simulink model "TractorEnergyComputation"  (R2025a)
settings: Solver=ode23t  StartTime=0.0  StopTime=2200  RelTol=1e-3  AbsTol=1e-3
InitFcn:
  | TractorEnergyComputationInput
undefined symbols (not defined in the file): engine, implement, pump, tc, tire, tk, tphi, tykc, tykphi, tyn
libraries: nesl_utility x32, fl_lib x18, sdl_lib x6, simulink x5
(part 2 of 2)

== system TractorEnergyComputation/Tractor/Tire RL ==
  S : Inport
  Bus Selector : BusSelector  OutputSignals=Rear Right Tire.tykc,Rear Right Tire.tykphi,Rear Right Tire.tyn,Rear Right Tire.tk,Rear Right Tire.tphi,Rear Right Tire.tc
  PS Add : fl_lib/Physical Signals/Functions/PS Add
  PS Gain : fl_lib/Physical Signals/Functions/PS Gain  gain=0.5
  Simulink-PS Converter : nesl_utility/Simulink-PS Converter  PhysicalDomain=network_engine_domain  SubClassName=ps_input  LeftPortType=input  RightPortType=output  PseudoPeriodic=off  Frequencies=[]  NoiseDistribution=none  NoiseParameters=[]  Unit=kN/m^2  AffineConversion=off  FilteringAndDerivatives=provide  SimscapeFilterOrder=1  InputFilterTimeConstant=0.001  UdotUserProvided=0
  Simulink-PS Converter1 : nesl_utility/Simulink-PS Converter  PhysicalDomain=network_engine_domain  SubClassName=ps_input  LeftPortType=input  RightPortType=output  PseudoPeriodic=off  Frequencies=[]  NoiseDistribution=none  NoiseParameters=[]  Unit=deg  AffineConversion=off  FilteringAndDerivatives=provide  SimscapeFilterOrder=1  InputFilterTimeConstant=0.001  UdotUserProvided=0
  Simulink-PS Converter2 : nesl_utility/Simulink-PS Converter  PhysicalDomain=network_engine_domain  SubClassName=ps_input  LeftPortType=input  RightPortType=output  PseudoPeriodic=off  Frequencies=[]  NoiseDistribution=none  NoiseParameters=[]  Unit=cm  AffineConversion=off  FilteringAndDerivatives=provide  SimscapeFilterOrder=1  InputFilterTimeConstant=0.001  UdotUserProvided=0
  Simulink-PS Converter3 : nesl_utility/Simulink-PS Converter  PhysicalDomain=network_engine_domain  SubClassName=ps_input  LeftPortType=input  RightPortType=output  PseudoPeriodic=off  Frequencies=[]  NoiseDistribution=none  NoiseParameters=[]  Unit=1  AffineConversion=off  FilteringAndDerivatives=provide  SimscapeFilterOrder=1  InputFilterTimeConstant=0.001  UdotUserProvided=0
  Simulink-PS Converter4 : nesl_utility/Simulink-PS Converter  PhysicalDomain=network_engine_domain  SubClassName=ps_input  LeftPortType=input  RightPortType=output  PseudoPeriodic=off  Frequencies=[]  NoiseDistribution=none  NoiseParameters=[]  Unit=1  AffineConversion=off  FilteringAndDerivatives=provide  SimscapeFilterOrder=1  InputFilterTimeConstant=0.001  UdotUserProvided=0
  Simulink-PS Converter5 : nesl_utility/Simulink-PS Converter  PhysicalDomain=network_engine_domain  SubClassName=ps_input  LeftPortType=input  RightPortType=output  PseudoPeriodic=off  Frequencies=[]  NoiseDistribution=none  NoiseParameters=[]  Unit=1  AffineConversion=off  FilteringAndDerivatives=provide  SimscapeFilterOrder=1  InputFilterTimeConstant=0.001  UdotUserProvided=0
  Tire RL : SimscapeComponentBlock  SourceFile=tire_soil  ComponentPath=tire_soil  ComponentVariants="[\"tire_soil\"]"  ComponentVariantNames="[\"tire_soil\"]"  ClassName=tire_soil  SchemaVersion=1  load_TLU=tire.loadVector kN  p_inflation_TLU=tire.inflationPressureVector kPa  deflection_TLU="tire.deflectionTable  cm"  area_TLU=tire.contactPatchArea cm^2  inflation_pressure=tire.inflationPressure kPa  k_e=tire.constructionCoefficient  r_e=tire.rollingRadiusRear m  bti=tire.sectionWidth m  hti=tire.sectionHeight m  model_compliance=sdl.enum.compliance.off  stiffness=1e6 N/m  damping=1000 N*s/m  model_inertia=sdl.enum.model_inertia.off  inertia=2 kg*m^2  initial_velocity=0 rad/s  vxlow=1 m/s  v_tr_thr=0.001 m/s  kpumin=-1.5  kpumax=1.5  p_thr=0.01 bar  b_thr=1 mm  r_e_t=0.5 m  rolling_radius_model=sdl.enum.RollingRadiusParameterization.Constant  fz0=4000 N  r_0=0.5 m  breff=8.39  dreff=0.26  freff=0.074  q_re0=0.99  q_v1=0.008  longvl=17 m/s  cz=5e5 N/m
      settings: CopyFcn=simscape.sscblock.internal.componentBlockCallback(gcbh,'COPY')  PreCopyFcn=simscape.sscblock.internal.componentBlockCallback(gcbh,'PRECOPY')  PreDeleteFcn=simscape.sscblock.internal.componentBlockCallback(gcbh,'PREDELETE')  InternalSimscapePortConfiguration="{\"Bottom\":[{\"id\":\"tykc\",\"label\":\"tykc\",\"type\":\"input\"},{\"id\":\"tykphi\",\"label\":\"tykphi\",\"type\":\"input\"},{\"id\":\"tyn\",\"label\":\"tyn\",\"type\":\"input\"}],\"Left\":[{\"id\":\"A\",\"label\":\"A\",\"type\":\"foundation.mechanical.rotational.rotational\"},{\"id\":\"H\",\"label\":\"H\",\"type\":\"foundation.mechanical.translational.translational\"}],\"Right\":[{\"id\":\"S\",\"label\":\"S\",\"type\":\"output\"}],\"Top\":[{\"id\":\"N\",\"label\":\"N\",\"type\":\"input\"},{\"id\":\"tc\",\"label\":\"tc\",\"type\":\"input\"},{\"id\":\"tphi\",\"label\":\"tphi\",\"type\":\"input\"},{\"id\":\"tk\",\"label\":\"tk\",\"type\":\"input\"}]}"
      mask Type: Tire (Tire-Soil)
  H : PMIOPort  Side=Left
  N : PMIOPort  Port=2  Side=Left
  VF : PMIOPort  Port=3  Side=Right
  RLT : PMIOPort  Port=4  Side=Right
  wires:
  S/1 -> Bus Selector/1
  Bus Selector/3 -> Simulink-PS Converter3/1  "<tyn>"
  Bus Selector/2 -> Simulink-PS Converter4/1  "<tykphi>"
  Bus Selector/4 -> Simulink-PS Converter2/1  "<tk>"
  Bus Selector/5 -> Simulink-PS Converter1/1  "<tphi>"
  Bus Selector/1 -> Simulink-PS Converter5/1  "<tykc>"
  Bus Selector/6 -> Simulink-PS Converter/1  "<tc>"
  connections:
  Simulink-PS Converter/RConn1 -- Tire RL/LConn4
  Simulink-PS Converter2/RConn1 -- Tire RL/LConn6
  Simulink-PS Converter1/RConn1 -- Tire RL/LConn5
  Simulink-PS Converter3/RConn1 -- Tire RL/RConn4
  Simulink-PS Converter5/RConn1 -- Tire RL/RConn2
  Simulink-PS Converter4/RConn1 -- Tire RL/RConn3
  PS Add/LConn1 -- N/RConn1
  VF/RConn1 -- PS Gain/LConn1
  PS Gain/RConn1 -- PS Add/LConn2
  PS Add/RConn1 -- Tire RL/LConn3
  RLT/RConn1 -- Tire RL/LConn1
  H/RConn1 -- Tire RL/LConn2

== system TractorEnergyComputation/Tractor/Tire RR ==
  S : Inport
  Bus Selector : BusSelector  OutputSignals=Rear Left Tire.tykc,Rear Left Tire.tykphi,Rear Left Tire.tyn,Rear Left Tire.tk,Rear Left Tire.tphi,Rear Left Tire.tc
  PS Add : fl_lib/Physical Signals/Functions/PS Add
  PS Gain : fl_lib/Physical Signals/Functions/PS Gain  gain=0.5
  Simulink-PS Converter : nesl_utility/Simulink-PS Converter  PhysicalDomain=network_engine_domain  SubClassName=ps_input  LeftPortType=input  RightPortType=output  PseudoPeriodic=off  Frequencies=[]  NoiseDistribution=none  NoiseParameters=[]  Unit=kN/m^2  AffineConversion=off  FilteringAndDerivatives=provide  SimscapeFilterOrder=1  InputFilterTimeConstant=0.001  UdotUserProvided=0
  Simulink-PS Converter1 : nesl_utility/Simulink-PS Converter  PhysicalDomain=network_engine_domain  SubClassName=ps_input  LeftPortType=input  RightPortType=output  PseudoPeriodic=off  Frequencies=[]  NoiseDistribution=none  NoiseParameters=[]  Unit=deg  AffineConversion=off  FilteringAndDerivatives=provide  SimscapeFilterOrder=1  InputFilterTimeConstant=0.001  UdotUserProvided=0
  Simulink-PS Converter2 : nesl_utility/Simulink-PS Converter  PhysicalDomain=network_engine_domain  SubClassName=ps_input  LeftPortType=input  RightPortType=output  PseudoPeriodic=off  Frequencies=[]  NoiseDistribution=none  NoiseParameters=[]  Unit=cm  AffineConversion=off  FilteringAndDerivatives=provide  SimscapeFilterOrder=1  InputFilterTimeConstant=0.001  UdotUserProvided=0
  Simulink-PS Converter3 : nesl_utility/Simulink-PS Converter  PhysicalDomain=network_engine_domain  SubClassName=ps_input  LeftPortType=input  RightPortType=output  PseudoPeriodic=off  Frequencies=[]  NoiseDistribution=none  NoiseParameters=[]  Unit=1  AffineConversion=off  FilteringAndDerivatives=provide  SimscapeFilterOrder=1  InputFilterTimeConstant=0.001  UdotUserProvided=0
  Simulink-PS Converter4 : nesl_utility/Simulink-PS Converter  PhysicalDomain=network_engine_domain  SubClassName=ps_input  LeftPortType=input  RightPortType=output  PseudoPeriodic=off  Frequencies=[]  NoiseDistribution=none  NoiseParameters=[]  Unit=1  AffineConversion=off  FilteringAndDerivatives=provide  SimscapeFilterOrder=1  InputFilterTimeConstant=0.001  UdotUserProvided=0
  Simulink-PS Converter5 : nesl_utility/Simulink-PS Converter  PhysicalDomain=network_engine_domain  SubClassName=ps_input  LeftPortType=input  RightPortType=output  PseudoPeriodic=off  Frequencies=[]  NoiseDistribution=none  NoiseParameters=[]  Unit=1  AffineConversion=off  FilteringAndDerivatives=provide  SimscapeFilterOrder=1  InputFilterTimeConstant=0.001  UdotUserProvided=0
  Tire RR : SimscapeComponentBlock  SourceFile=tire_soil  ComponentPath=tire_soil  ComponentVariants="[\"tire_soil\"]"  ComponentVariantNames="[\"tire_soil\"]"  ClassName=tire_soil  SchemaVersion=1  load_TLU=tire.loadVector kN  p_inflation_TLU=tire.inflationPressureVector kPa  deflection_TLU=tire.deflectionTable cm  area_TLU=tire.contactPatchArea cm^2  inflation_pressure=tire.inflationPressure kPa  k_e=tire.constructionCoefficient  r_e=tire.rollingRadiusRear m  bti=tire.sectionWidth m  hti=tire.sectionHeight m  model_compliance=sdl.enum.compliance.off  stiffness=1e6 N/m  damping=1000 N*s/m  model_inertia=sdl.enum.model_inertia.off  inertia=2 kg*m^2  initial_velocity=0 rad/s  vxlow=1 m/s  v_tr_thr=0.001 m/s  kpumin=-1.5  kpumax=1.5  p_thr=0.01 bar  b_thr=1 mm  r_e_t=0.5 m  rolling_radius_model=sdl.enum.RollingRadiusParameterization.Constant  fz0=4000 N  r_0=0.5 m  breff=8.39  dreff=0.26  freff=0.074  q_re0=0.99  q_v1=0.008  longvl=17 m/s  cz=5e5 N/m
      settings: CopyFcn=simscape.sscblock.internal.componentBlockCallback(gcbh,'COPY')  PreCopyFcn=simscape.sscblock.internal.componentBlockCallback(gcbh,'PRECOPY')  PreDeleteFcn=simscape.sscblock.internal.componentBlockCallback(gcbh,'PREDELETE')  InternalSimscapePortConfiguration="{\"Bottom\":[{\"id\":\"tykc\",\"label\":\"tykc\",\"type\":\"input\"},{\"id\":\"tykphi\",\"label\":\"tykphi\",\"type\":\"input\"},{\"id\":\"tyn\",\"label\":\"tyn\",\"type\":\"input\"}],\"Left\":[{\"id\":\"A\",\"label\":\"A\",\"type\":\"foundation.mechanical.rotational.rotational\"},{\"id\":\"H\",\"label\":\"H\",\"type\":\"foundation.mechanical.translational.translational\"}],\"Right\":[{\"id\":\"S\",\"label\":\"S\",\"type\":\"output\"}],\"Top\":[{\"id\":\"N\",\"label\":\"N\",\"type\":\"input\"},{\"id\":\"tc\",\"label\":\"tc\",\"type\":\"input\"},{\"id\":\"tphi\",\"label\":\"tphi\",\"type\":\"input\"},{\"id\":\"tk\",\"label\":\"tk\",\"type\":\"input\"}]}"
      mask Type: Tire (Tire-Soil)
  N : PMIOPort  Side=Left
  H : PMIOPort  Port=2  Side=Left
  RRT : PMIOPort  Port=3  Side=Left
  VF : PMIOPort  Port=4  Side=Right
  wires:
  S/1 -> Bus Selector/1
  Bus Selector/6 -> Simulink-PS Converter/1  "<tc>"
  Bus Selector/1 -> Simulink-PS Converter5/1  "<tykc>"
  Bus Selector/2 -> Simulink-PS Converter4/1  "<tykphi>"
  Bus Selector/3 -> Simulink-PS Converter3/1  "<tyn>"
  Bus Selector/4 -> Simulink-PS Converter2/1  "<tk>"
  Bus Selector/5 -> Simulink-PS Converter1/1  "<tphi>"
  connections:
  Simulink-PS Converter/RConn1 -- Tire RR/LConn4
  Simulink-PS Converter1/RConn1 -- Tire RR/LConn5
  Simulink-PS Converter2/RConn1 -- Tire RR/LConn6
  Simulink-PS Converter3/RConn1 -- Tire RR/RConn4
  Simulink-PS Converter4/RConn1 -- Tire RR/RConn3
  Simulink-PS Converter5/RConn1 -- Tire RR/RConn2
  PS Gain/RConn1 -- PS Add/LConn2
  N/RConn1 -- PS Add/LConn1
  VF/RConn1 -- PS Gain/LConn1
  PS Add/RConn1 -- Tire RR/LConn3
  RRT/RConn1 -- Tire RR/LConn1
  H/RConn1 -- Tire RR/LConn2

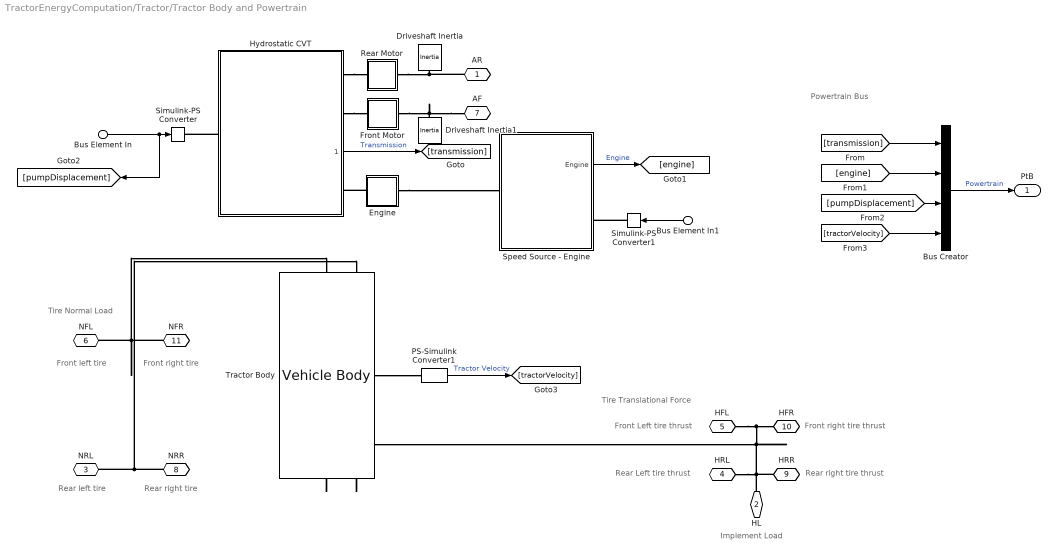
== system TractorEnergyComputation/Tractor/Tractor Body and Powertrain ==
  note: Powertrain Bus
  note: Tire Normal Load
  note: Tire Translational Force
  note: Front right tire thrust
  note: Rear right tire thrust
  note: Front Left tire thrust
  note: Rear Left tire thrust
  note: Front right tire
  note: Rear left tire
  note: Front left tire
  note: Rear right tire
  note: Implement Load
  Bus Element In : Inport  PortName=C  Element=Pump Displacement
  Bus Element In1 : Inport  PortName=C  Element=Speed Command
  Bus Creator : BusCreator  Inputs=4
  Driveshaft Inertia : fl_lib/Mechanical/Rotational Elements/Inertia  inertia=finalDrive.inertiaDriveshaft kg*m^2  num_ports=foundation.enum.numPorts2.one  w_specify=on  w_priority=None  w=0 rpm  w_nominal_specify=off  w_nominal_value=1  w_nominal_unit=rad/s  t_specify=off  t_priority=High  t=0 N*m  t_nominal_specify=off  t_nominal_value=1  t_nominal_unit=N*m
  Driveshaft Inertia1 : fl_lib/Mechanical/Rotational Elements/Inertia  inertia=finalDrive.inertiaDriveshaft kg*m^2  num_ports=foundation.enum.numPorts2.one  w_specify=on  w_priority=None  w=0 rpm  w_nominal_specify=off  w_nominal_value=1  w_nominal_unit=rad/s  t_specify=off  t_priority=High  t=0 N*m  t_nominal_specify=off  t_nominal_value=1  t_nominal_unit=N*m
  Engine : Subsystem
      settings: PortSchema="{\"entries\":[{\"content\":{\"sides\":[{\"content\":{},\"type\":\"ConnectorPlacement.EquallySpacedRectSide\",\"uuid\":\"92eebf28-269a-4925-a955-a9d1c44b965b\"},{\"content\":{\"side\":\"RIGHT\"},\"type\":\"ConnectorPlacement.EquallySpacedRectSide\",\"uuid\":\"c7d6808e-0022-4ac6-baaf-1452e02bfec1\"},{\"content\":{\"connectorIds\":[\"LConn1\"],\"side\":\"TOP\"},\"type\":\"ConnectorPlacement.EquallySpacedRectSide\",\"uuid\":\"598768ff-2342-4a1c-9a1c-354d4df076d5\"},{\"content\":{\"connectorIds\":[\"RConn1\"],\"side\":\"BOTTOM\"},\"type\":\"ConnectorPlacement.EquallySpacedRectSide\",\"uuid\":\"a8e2d810-51b4-480a-8888-7fbba5dd7c90\"}]},\"type\":\"ConnectorPlacement.EquallySpacedConnector\",\"uuid\":\"c2f50c2b-379b-41d6-9ef6-b6270bc7ebba\"}],\"packageUris\":[\"http://schema.mathworks.com/mf0/Connector/R2020b\"],\"version\":\"1.0\"}"
  Front Motor : Subsystem
      settings: PortSchema="{\"entries\":[{\"content\":{\"sides\":[{\"content\":{},\"type\":\"ConnectorPlacement.EquallySpacedRectSide\",\"uuid\":\"92eebf28-269a-4925-a955-a9d1c44b965b\"},{\"content\":{\"side\":\"RIGHT\"},\"type\":\"ConnectorPlacement.EquallySpacedRectSide\",\"uuid\":\"c7d6808e-0022-4ac6-baaf-1452e02bfec1\"},{\"content\":{\"connectorIds\":[\"LConn1\"],\"side\":\"TOP\"},\"type\":\"ConnectorPlacement.EquallySpacedRectSide\",\"uuid\":\"598768ff-2342-4a1c-9a1c-354d4df076d5\"},{\"content\":{\"connectorIds\":[\"RConn1\"],\"side\":\"BOTTOM\"},\"type\":\"ConnectorPlacement.EquallySpacedRectSide\",\"uuid\":\"a8e2d810-51b4-480a-8888-7fbba5dd7c90\"}]},\"type\":\"ConnectorPlacement.EquallySpacedConnector\",\"uuid\":\"c2f50c2b-379b-41d6-9ef6-b6270bc7ebba\"}],\"packageUris\":[\"http://schema.mathworks.com/mf0/Connector/R2020b\"],\"version\":\"1.0\"}"
  Hydrostatic CVT : Subsystem  ReferencedSubsystem=HydrostaticCVT
      settings: PortSchema="{\"entries\":[{\"content\":{\"sides\":[{\"content\":{\"connectorIds\":[\"LConn2\"]},\"type\":\"ConnectorPlacement.EquallySpacedRectSide\",\"uuid\":\"e98c307e-384f-4f6d-84ec-b1e3747c2742\"},{\"content\":{\"connectorIds\":[\"RConn1\",\"RConn2\",\"Out1\",\"LConn1\"],\"side\":\"RIGHT\"},\"type\":\"ConnectorPlacement.EquallySpacedRectSide\",\"uuid\":\"8cf92fb4-b64d-4865-8313-0964738a3102\"},{\"content\":{\"side\":\"TOP\"},\"type\":\"ConnectorPlacement.EquallySpacedRectSide\",\"uuid\":\"5529046d-fa81-4c87-9e58-4bcc6f8343df\"},{\"content\":{\"side\":\"BOTTOM\"},\"type\":\"ConnectorPlacement.EquallySpacedRectSide\",\"uuid\":\"0f2d78cd-5597-48dc-a814-c7cd3f15dde1\"}]},\"type\":\"ConnectorPlacement.EquallySpacedConnector\",\"uuid\":\"d1cf8514-964a-4874-a812-4541b3ddd120\"}],\"packageUris\":[\"http://schema.mathworks.com/mf0/Connector/R2020b\"],\"version\":\"1.0\"}"
  PS-Simulink Converter1 : nesl_utility/PS-Simulink Converter  PhysicalDomain=network_engine_domain  SubClassName=ps_output  LeftPortType=input  RightPortType=output  PseudoPeriodic=off  Frequencies=[]  VectorFormat=1-D array  Unit=km/hr  AffineConversion=off
  Rear Motor : Subsystem
      settings: PortSchema="{\"entries\":[{\"content\":{\"sides\":[{\"content\":{},\"type\":\"ConnectorPlacement.EquallySpacedRectSide\",\"uuid\":\"92eebf28-269a-4925-a955-a9d1c44b965b\"},{\"content\":{\"side\":\"RIGHT\"},\"type\":\"ConnectorPlacement.EquallySpacedRectSide\",\"uuid\":\"c7d6808e-0022-4ac6-baaf-1452e02bfec1\"},{\"content\":{\"connectorIds\":[\"LConn1\"],\"side\":\"TOP\"},\"type\":\"ConnectorPlacement.EquallySpacedRectSide\",\"uuid\":\"598768ff-2342-4a1c-9a1c-354d4df076d5\"},{\"content\":{\"connectorIds\":[\"RConn1\"],\"side\":\"BOTTOM\"},\"type\":\"ConnectorPlacement.EquallySpacedRectSide\",\"uuid\":\"a8e2d810-51b4-480a-8888-7fbba5dd7c90\"}]},\"type\":\"ConnectorPlacement.EquallySpacedConnector\",\"uuid\":\"c2f50c2b-379b-41d6-9ef6-b6270bc7ebba\"}],\"packageUris\":[\"http://schema.mathworks.com/mf0/Connector/R2020b\"],\"version\":\"1.0\"}"
  Simulink-PS Converter : nesl_utility/Simulink-PS Converter  PhysicalDomain=network_engine_domain  SubClassName=ps_input  LeftPortType=input  RightPortType=output  PseudoPeriodic=off  Frequencies=[]  NoiseDistribution=none  NoiseParameters=[]  Unit=cm^3/rev  AffineConversion=off  FilteringAndDerivatives=provide  SimscapeFilterOrder=1  InputFilterTimeConstant=0.001  UdotUserProvided=0
  Simulink-PS Converter1 : nesl_utility/Simulink-PS Converter  PhysicalDomain=network_engine_domain  SubClassName=ps_input  LeftPortType=input  RightPortType=output  PseudoPeriodic=off  Frequencies=[]  NoiseDistribution=none  NoiseParameters=[]  Unit=rpm  AffineConversion=off  FilteringAndDerivatives=provide  SimscapeFilterOrder=1  InputFilterTimeConstant=0.001  UdotUserProvided=0
  Speed Source - Engine : Subsystem
      settings: PortSchema="{\"entries\":[{\"content\":{\"sides\":[{\"content\":{\"connectorIds\":[\"Out1\",\"LConn1\"]},\"type\":\"ConnectorPlacement.EquallySpacedRectSide\",\"uuid\":\"893d34ea-3b68-4e33-a67a-452726c44412\"},{\"content\":{\"connectorIds\":[\"RConn1\"],\"side\":\"RIGHT\"},\"type\":\"ConnectorPlacement.EquallySpacedRectSide\",\"uuid\":\"36b2695b-8811-427c-b3d4-10ce1d3bb3e5\"},{\"content\":{\"side\":\"TOP\"},\"type\":\"ConnectorPlacement.EquallySpacedRectSide\",\"uuid\":\"39e3a5de-3435-43d6-80cb-ad06275add25\"}]},\"type\":\"ConnectorPlacement.EquallySpacedConnector\",\"uuid\":\"b2b9cbdb-1a63-4aca-a9b5-b09fdbada543\"}],\"packageUris\":[\"http://schema.mathworks.com/mf0/Connector/R2020b\"],\"version\":\"1.0\"}"
  Tractor Body : sdl_lib/Tires & Vehicles/Vehicle Body  mass=driveline.massTractor kg  n_w=driveline.nWheelsPerAxle  x_f=driveline.distanceFrontAxleCG m  x_r=driveline.distanceRearAxleCG m  y_c=driveline.heightCG m  mass_var=simscape.enum.onoff.off  g=9.81 m/s^2  liftoff_warning=simscape.enum.onoff.off  area=driveline.areaFrontal m^2  Cd_var=false  Cd=driveline.coefficientDrag  rho=driveline.densityAir kg/m^3  model_pitch=simscape.enum.onoff.off  inertia=4000 kg*m^2  suspension_model=sdl.enum.linearTLU.linear  k_f=1e4 N/m  b_f=1e4 N/(m/s)  k_r=1e4 N/m  b_r=1e4 N/(m/s)  k_f_TLU=[-2000, -1000, 0, 1000, 2000] N  x_f_TLU=[-.4, -.2, 0, .2, .4] m  b_f_TLU=[-200, -100, 0, 100, 200] N  v_f_TLU=[-4, -2, 0, 2, 4] m/s  k_r_TLU=[-2000, -1000, 0, 1000, 2000] N  x_r_TLU=[-.4, -.2, 0, .2, .4] m  b_r_TLU=[-200, -100, 0, 100, 200] N  v_r_TLU=[-4, -2, 0, 2, 4] m/s  interp_method=simscape.enum.interpolation.linear  extrap_method=simscape.enum.extrapolation.linear  model_hardstop=simscape.enum.onoff.off  upper_bound_f=.25 m  lower_bound_f=-.25 m  stop_k_f=1e6 N/m  stop_b_f=150 N/(m/s)  upper_bound_r=.25 m  lower_bound_r=-.25 m  stop_k_r=1e6 N/m  stop_b_r=150 N/(m/s)  initial_pitch=0 rad  initial_pitch_rate=0 rad/s  v_specify=off  v_priority=High  v=0 m/s  v_nominal_specify=off  v_nominal_value=1  v_nominal_unit=m/s
      settings: InternalSimscapePortConfiguration="{\"Bottom\":[{\"id\":\"NR\",\"label\":\"NR\",\"type\":\"output\"},{\"id\":\"NF\",\"label\":\"NF\",\"type\":\"output\"},{\"id\":\"beta\",\"label\":\"beta\",\"type\":\"input\"}],\"Left\":[{\"id\":\"H\",\"label\":\"H\",\"type\":\"foundation.mechanical.translational.translational\"}],\"Right\":[],\"Top\":[{\"id\":\"V\",\"label\":\"V\",\"type\":\"output\"},{\"id\":\"wind\",\"label\":\"W\",\"type\":\"input\"}]}"
  AR : PMIOPort  Side=Left
  HL : PMIOPort  Port=2  Side=Left
  NRL : PMIOPort  Port=3  Side=Left
  HRL : PMIOPort  Port=4  Side=Left
  HFL : PMIOPort  Port=5  Side=Left
  NFL : PMIOPort  Port=6  Side=Left
  "AF " : PMIOPort  Port=7  Side=Right
  NRR : PMIOPort  Port=8  Side=Right
  HRR : PMIOPort  Port=9  Side=Right
  HFR : PMIOPort  Port=10  Side=Right
  NFR : PMIOPort  Port=11  Side=Right
  PtB : Outport
  wires:
  PS-Simulink Converter1/1 -> [tractorVelocity]  "Tractor Velocity"
  Hydrostatic CVT/1 -> [transmission]  "Transmission"
  Speed Source - Engine/1(Engine) -> [engine]  "Engine"
  Bus Creator/1 -> PtB/1  "Powertrain"
  [transmission] -> Bus Creator/1
  [engine] -> Bus Creator/2
  [pumpDisplacement] -> Bus Creator/3
  [tractorVelocity] -> Bus Creator/4
  Bus Element In/1 -> [pumpDisplacement], Simulink-PS Converter/1
  Bus Element In1/1 -> Simulink-PS Converter1/1
  connections:
  HRL/RConn1 -- HL/RConn1 -- HRR/RConn1 -- HFL/RConn1 -- HFR/RConn1 -- Tractor Body/LConn1
  AR/RConn1 -- Rear Motor/RConn1 -- Driveshaft Inertia/LConn1
  Engine/LConn1 -- Speed Source - Engine/RConn1
  NRR/RConn1 -- Tractor Body/RConn1 -- NRL/RConn1
  NFR/RConn1 -- Tractor Body/RConn2 -- NFL/RConn1
  Tractor Body/LConn2 -- PS-Simulink Converter1/LConn1
  Hydrostatic CVT/LConn2 -- Simulink-PS Converter/RConn1
  "AF "/RConn1 -- Front Motor/RConn1 -- Driveshaft Inertia1/LConn1
  Simulink-PS Converter1/RConn1 -- Speed Source - Engine/LConn1
  Hydrostatic CVT/RConn1 -- Rear Motor/LConn1
  Hydrostatic CVT/RConn2 -- Front Motor/LConn1
  Engine/RConn1 -- Hydrostatic CVT/LConn1

== system TractorEnergyComputation/System Signals and Information/Power and Energy Calculations/Charge Pump Computation ==
  System Bus : Inport
  Bus Selector : BusSelector  OutputSignals=Engine.engineSpeed,Transmission.Charge Pump.trq (N*m),Pump Displacement
  Bus Selector1 : BusSelector  OutputSignals=Pump Displacement,Transmission.Charge Pump.q (m^3/s),Transmission.Charge Pump.P (bar)
  Charge Pump Input Energy Computation : Subsystem
  Charge Pump Output Energy Computation : Subsystem
  Sump open pressure : Constant  Value=1.01325
  Input Energy : Outport
  "Output Energy " : Outport  Port=2
  Input Power : Outport  Port=3
  Output Power : Outport  Port=4
  wires:
  Charge Pump Output Energy Computation/1(Output Energy) -> "Output Energy "/1
  Charge Pump Input Energy Computation/1(Input Energy) -> Input Energy/1
  Bus Selector1/3 -> Charge Pump Output Energy Computation/3(pressureB (bar))  "<P (bar)>"
  Bus Selector1/2 -> Charge Pump Output Energy Computation/2(pumpFlow (m^3/s))  "<q (m^3/s)>"
  Bus Selector1/1 -> Charge Pump Output Energy Computation/1(dispPump (cm^3/rev))  "<Pump Displacement>"
  Bus Selector/3 -> Charge Pump Input Energy Computation/3(dispPump (cm^3/rev))  "<Pump Displacement>"
  Bus Selector/2 -> Charge Pump Input Energy Computation/2(tPump (N*m))  "<trq (N*m)>"
  Bus Selector/1 -> Charge Pump Input Energy Computation/1(wEngine (rpm))  "<engineSpeed>"
  System Bus/1 -> Bus Selector/1, Bus Selector1/1
  Sump open pressure/1 -> Charge Pump Output Energy Computation/4(pressureA (bar))
  Charge Pump Input Energy Computation/2(Input Power) -> Input Power/1
  Charge Pump Output Energy Computation/2(Output Power) -> Output Power/1

== system TractorEnergyComputation/System Signals and Information/Power and Energy Calculations/Front Motor Computation ==
  System Bus : Inport
  Bus Selector : BusSelector  OutputSignals=Transmission.Front Motor.w (rpm),Transmission.Front Motor.trq (N*m),Pump Displacement
  Bus Selector1 : BusSelector  OutputSignals=Pump Displacement,Transmission.Front Motor.q (m^3/s),Transmission.Pipe A.pB (bar),Transmission.Pipe B.pB (bar)
  Motor Input Energy Computation : Subsystem
  Motor Output Energy Computation : Subsystem
  Output Energy : Outport
  "Input Energy " : Outport  Port=2
  Output Power : Outport  Port=3
  Input Power : Outport  Port=4
  wires:
  Bus Selector1/4 -> Motor Input Energy Computation/4(pressureB (bar))  "<pB (bar)>"
  Bus Selector1/3 -> Motor Input Energy Computation/3(pressureA (bar))  "<pB (bar)>"
  Bus Selector1/2 -> Motor Input Energy Computation/2(motorFlow (m^3/s))  "<q (m^3/s)>"
  Bus Selector1/1 -> Motor Input Energy Computation/1(dispPump (cm^3/rev))  "<Pump Displacement>"
  Bus Selector/1 -> Motor Output Energy Computation/1(wTransmission (rpm))  "<w (rpm)>"
  Bus Selector/3 -> Motor Output Energy Computation/3(dispPump (cm^3/rev))  "<Pump Displacement>"
  Bus Selector/2 -> Motor Output Energy Computation/2(tTransmission (N*m))  "<trq (N*m)>"
  System Bus/1 -> Bus Selector/1, Bus Selector1/1
  Motor Input Energy Computation/1("Input Energy ") -> "Input Energy "/1
  Motor Output Energy Computation/1(Output Energy) -> Output Energy/1
  Motor Output Energy Computation/2(Output Power) -> Output Power/1
  Motor Input Energy Computation/2(Input Power) -> Input Power/1

== system TractorEnergyComputation/System Signals and Information/Power and Energy Calculations/Pump Computation ==
  System Bus : Inport
  Bus Selector : BusSelector  OutputSignals=Engine.engineSpeed,Transmission.Main Pump.trq (N*m),Pump Displacement
  Bus Selector1 : BusSelector  OutputSignals=Pump Displacement,Transmission.Main Pump.q (m^3/s),Transmission.Pipe B.pA (bar),Transmission.Pipe A.pA (bar)
  Pump Input Energy Computation : Subsystem
  Pump Output Energy Computation : Subsystem
  Input Energy : Outport
  "Output Energy " : Outport  Port=2
  Input Power : Outport  Port=3
  Output Power : Outport  Port=4
  wires:
  System Bus/1 -> Bus Selector1/1, Bus Selector/1
  Bus Selector/1 -> Pump Input Energy Computation/1(wEngine (rpm))  "<engineSpeed>"
  Bus Selector/2 -> Pump Input Energy Computation/2(tPump (N*m))  "<trq (N*m)>"
  Bus Selector/3 -> Pump Input Energy Computation/3(dispPump (cm^3/rev))  "<Pump Displacement>"
  Bus Selector1/1 -> Pump Output Energy Computation/1(dispPump (cm^3/rev))  "<Pump Displacement>"
  Bus Selector1/2 -> Pump Output Energy Computation/2(pumpFlow (m^3/s))  "<q (m^3/s)>"
  Bus Selector1/3 -> Pump Output Energy Computation/3(pressureA (bar))  "<pA (bar)>"
  Bus Selector1/4 -> Pump Output Energy Computation/4(pressureB (bar))  "<pA (bar)>"
  Pump Input Energy Computation/1(Input Energy) -> Input Energy/1
  Pump Output Energy Computation/1(Output Energy) -> "Output Energy "/1
  Pump Input Energy Computation/2(Input Power) -> Input Power/1
  Pump Output Energy Computation/2(Output Power) -> Output Power/1

== system TractorEnergyComputation/System Signals and Information/Power and Energy Calculations/Rear Motor Computation ==
  System Bus : Inport
  Bus Selector : BusSelector  OutputSignals=Transmission.Rear Motor.w (rpm),Transmission.Rear Motor.trq (N*m),Pump Displacement
  Bus Selector1 : BusSelector  OutputSignals=Pump Displacement,Transmission.Rear Motor.q (m^3/s),Transmission.Pipe A.pB (bar),Transmission.Pipe B.pB (bar)
  Motor Input Energy Computation : Subsystem
  Motor Output Energy Computation : Subsystem
  Output Energy : Outport
  "Input Energy  " : Outport  Port=2
  Output Power : Outport  Port=3
  Input Power : Outport  Port=4
  wires:
  Motor Output Energy Computation/1(Output Energy) -> Output Energy/1
  Motor Input Energy Computation/1("Input Energy ") -> "Input Energy  "/1
  System Bus/1 -> Bus Selector1/1, Bus Selector/1
  Bus Selector/2 -> Motor Output Energy Computation/2(tTransmission (N*m))  "<trq (N*m)>"
  Bus Selector/3 -> Motor Output Energy Computation/3(dispPump (cm^3/rev))  "<Pump Displacement>"
  Bus Selector/1 -> Motor Output Energy Computation/1(wTransmission (rpm))  "<w (rpm)>"
  Bus Selector1/1 -> Motor Input Energy Computation/1(dispPump (cm^3/rev))  "<Pump Displacement>"
  Bus Selector1/2 -> Motor Input Energy Computation/2(motorFlow (m^3/s))  "<q (m^3/s)>"
  Bus Selector1/3 -> Motor Input Energy Computation/3(pressureA (bar))  "<pB (bar)>"
  Bus Selector1/4 -> Motor Input Energy Computation/4(pressureB (bar))  "<pB (bar)>"
  Motor Output Energy Computation/2(Output Power) -> Output Power/1
  Motor Input Energy Computation/2(Input Power) -> Input Power/1

== system TractorEnergyComputation/System Signals and Information/Power and Energy Calculations/Relief Valve A Computation ==
  System Bus : Inport
  Abs : Abs  ZeroCross=off  SaturateOnIntegerOverflow=off
  Abs1 : Abs  ZeroCross=off  SaturateOnIntegerOverflow=off
  Add1 : Sum  Inputs=+-
  Add2 : Sum  Inputs=+-
  Bus Selector : BusSelector  OutputSignals=Transmission.Pipe A.pB (bar),Transmission.Flow Relief A.q (m^3/s),Transmission.Pipe B.pB (bar)
  Gain1 : Gain  Gain=1e5
  Gain2 : Gain  Gain=1e5
  Integrator : Integrator
  Integrator1 : Integrator
  Product : Product
  Product1 : Product
  convert to kW : Gain  Gain=1e-3
  convert to kW1 : Gain  Gain=1e-3
  "Energy Loss " : Outport
  Power Loss : Outport  Port=2
  wires:
  Gain2/1 -> Abs/1
  Product/1 -> Gain2/1
  Product1/1 -> Gain1/1
  Gain1/1 -> Abs1/1
  Abs/1 -> convert to kW/1
  Abs1/1 -> convert to kW1/1
  Integrator/1 -> Add1/1  "Relief A Inlet Energy"
  Integrator1/1 -> Add1/2  "Relief A Outlet Energy"
  Add1/1 -> "Energy Loss "/1  "Energy Loss Relief Valve A"
  convert to kW/1 -> Add2/1, Integrator/1
  convert to kW1/1 -> Add2/2, Integrator1/1
  System Bus/1 -> Bus Selector/1
  Bus Selector/1 -> Product/1  "<pB (bar)>"
  Bus Selector/2 -> Product1/1, Product/2  "<q (m^3/s)>"
  Bus Selector/3 -> Product1/2  "<pB (bar)>"
  Add2/1 -> Power Loss/1  "Power Loss Relief Valve A"

== system TractorEnergyComputation/System Signals and Information/Power and Energy Calculations/Relief Valve B Computation ==
  System Bus : Inport
  Abs : Abs  ZeroCross=off  SaturateOnIntegerOverflow=off
  Abs1 : Abs  ZeroCross=off  SaturateOnIntegerOverflow=off
  Add1 : Sum  Inputs=-+
  Add2 : Sum  Inputs=-+
  Bus Selector : BusSelector  OutputSignals=Transmission.Pipe A.pB (bar),Transmission.Flow Relief B.q (m^3/s),Transmission.Pipe B.pB (bar)
  Gain1 : Gain  Gain=1e5
  Gain2 : Gain  Gain=1e5
  Integrator : Integrator
  Integrator1 : Integrator
  Product : Product
  Product1 : Product
  convert to kW : Gain  Gain=1e-3
  convert to kW1 : Gain  Gain=1e-3
  "Energy Loss " : Outport
  "Power Loss " : Outport  Port=2
  wires:
  Add1/1 -> "Energy Loss "/1  "Energy Loss Relief Valve B"
  Integrator1/1 -> Add1/2  "Relief B Inlet Energy"
  Integrator/1 -> Add1/1  "Relief B Outlet Energy"
  Abs1/1 -> convert to kW1/1
  Abs/1 -> convert to kW/1
  Gain1/1 -> Abs1/1
  Gain2/1 -> Abs/1
  convert to kW/1 -> Add2/1, Integrator/1
  System Bus/1 -> Bus Selector/1
  Bus Selector/1 -> Product/1  "<pB (bar)>"
  Bus Selector/3 -> Product1/2  "<pB (bar)>"
  Bus Selector/2 -> Product/2, Product1/1  "<q (m^3/s)>"
  Product/1 -> Gain2/1
  Product1/1 -> Gain1/1
  convert to kW1/1 -> Add2/2, Integrator1/1
  Add2/1 -> "Power Loss "/1  "Power Loss Relief Valve B"

== system TractorEnergyComputation/Tractor/Tractor Body and Powertrain/Engine ==
  Mechanical Rotational Reference : fl_lib/Mechanical/Rotational Elements/Mechanical Rotational Reference
  PS Terminator : fl_lib/Physical Signals/Sinks/PS Terminator
  Rotational Power Sensor : sdl_lib/Sensors/Rotational Power Sensor  measurement_type=sdl.enum.rotationalPowerSensorType.instantaneous  averaging_period=1 s  max_frequency=1000 Hz  max_speed=1000 rpm
      settings: InternalSimscapePortConfiguration="{\"Bottom\":[],\"Left\":[{\"id\":\"S\",\"label\":\"S\",\"type\":\"foundation.mechanical.rotational.rotational\"},{\"id\":\"R\",\"label\":\"R\",\"type\":\"foundation.mechanical.rotational.rotational\"},{\"id\":\"C\",\"label\":\"C\",\"type\":\"foundation.mechanical.rotational.rotational\"}],\"Right\":[{\"id\":\"P\",\"label\":\"P\",\"type\":\"output\"}],\"Top\":[]}"
  S : PMIOPort  Side=Left
  R : PMIOPort  Port=2  Side=Right
  connections:
  Rotational Power Sensor/RConn1 -- PS Terminator/LConn1
  Rotational Power Sensor/LConn3 -- Mechanical Rotational Reference/LConn1
  S/RConn1 -- Rotational Power Sensor/LConn1
  R/RConn1 -- Rotational Power Sensor/LConn2

== system TractorEnergyComputation/Tractor/Tractor Body and Powertrain/Front Motor ==
  Mechanical Rotational Reference : fl_lib/Mechanical/Rotational Elements/Mechanical Rotational Reference
  PS Terminator : fl_lib/Physical Signals/Sinks/PS Terminator
  Rotational Power Sensor : sdl_lib/Sensors/Rotational Power Sensor  measurement_type=sdl.enum.rotationalPowerSensorType.instantaneous  averaging_period=1 s  max_frequency=1000 Hz  max_speed=1000 rpm
      settings: InternalSimscapePortConfiguration="{\"Bottom\":[],\"Left\":[{\"id\":\"S\",\"label\":\"S\",\"type\":\"foundation.mechanical.rotational.rotational\"},{\"id\":\"R\",\"label\":\"R\",\"type\":\"foundation.mechanical.rotational.rotational\"},{\"id\":\"C\",\"label\":\"C\",\"type\":\"foundation.mechanical.rotational.rotational\"}],\"Right\":[{\"id\":\"P\",\"label\":\"P\",\"type\":\"output\"}],\"Top\":[]}"
  S : PMIOPort  Side=Left
  R : PMIOPort  Port=2  Side=Right
  connections:
  R/RConn1 -- Rotational Power Sensor/LConn2
  S/RConn1 -- Rotational Power Sensor/LConn1
  Rotational Power Sensor/LConn3 -- Mechanical Rotational Reference/LConn1
  Rotational Power Sensor/RConn1 -- PS Terminator/LConn1

== system TractorEnergyComputation/Tractor/Tractor Body and Powertrain/Rear Motor ==
  Mechanical Rotational Reference : fl_lib/Mechanical/Rotational Elements/Mechanical Rotational Reference
  PS Terminator : fl_lib/Physical Signals/Sinks/PS Terminator
  Rotational Power Sensor : sdl_lib/Sensors/Rotational Power Sensor  measurement_type=sdl.enum.rotationalPowerSensorType.instantaneous  averaging_period=1 s  max_frequency=1000 Hz  max_speed=1000 rpm
      settings: InternalSimscapePortConfiguration="{\"Bottom\":[],\"Left\":[{\"id\":\"S\",\"label\":\"S\",\"type\":\"foundation.mechanical.rotational.rotational\"},{\"id\":\"R\",\"label\":\"R\",\"type\":\"foundation.mechanical.rotational.rotational\"},{\"id\":\"C\",\"label\":\"C\",\"type\":\"foundation.mechanical.rotational.rotational\"}],\"Right\":[{\"id\":\"P\",\"label\":\"P\",\"type\":\"output\"}],\"Top\":[]}"
  S : PMIOPort  Side=Left
  R : PMIOPort  Port=2  Side=Right
  connections:
  Rotational Power Sensor/RConn1 -- PS Terminator/LConn1
  Rotational Power Sensor/LConn3 -- Mechanical Rotational Reference/LConn1
  S/RConn1 -- Rotational Power Sensor/LConn1
  R/RConn1 -- Rotational Power Sensor/LConn2

== system TractorEnergyComputation/Tractor/Tractor Body and Powertrain/Speed Source - Engine ==
  note: This tractor engine operates ar fixed speed through governor control for agriculture hydraulic equipment requirement.
      | The governor controls the fuel injection into the cylinders to maintain
      | speed constant to compensate for load.
  Ideal Angular Velocity Source : fl_lib/Mechanical/Mechanical Sources/Ideal Angular Velocity Source
  Mechanical Rotational Reference : fl_lib/Mechanical/Rotational Elements/Mechanical Rotational Reference
  Sensor Engine : Subsystem
      mask Display: disp('S')
  SC : PMIOPort  Side=Left
  Shaft : PMIOPort  Port=2  Side=Right
  Engine : Outport
  wires:
  Sensor Engine/1(engine) -> Engine/1
  connections:
  Mechanical Rotational Reference/LConn1 -- Ideal Angular Velocity Source/RConn2
  Ideal Angular Velocity Source/LConn1 -- Sensor Engine/LConn1
  Sensor Engine/RConn1 -- Shaft/RConn1
  Ideal Angular Velocity Source/RConn1 -- SC/RConn1

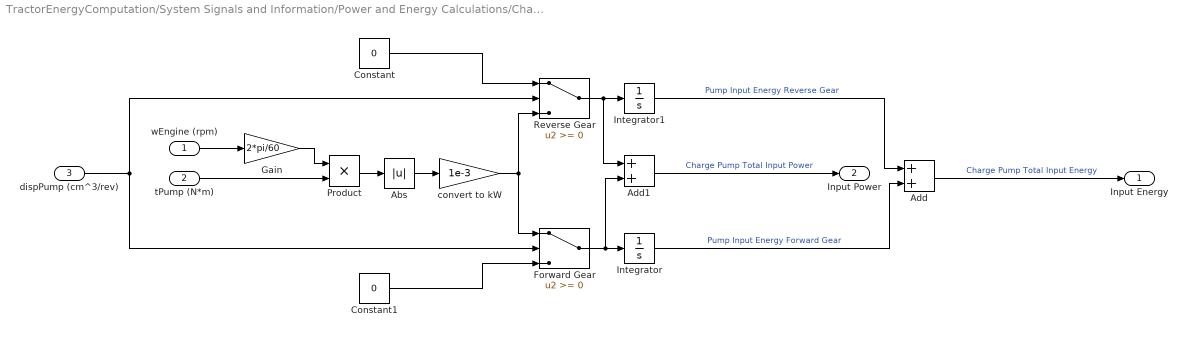
== system TractorEnergyComputation/System Signals and Information/Power and Energy Calculations/Charge Pump Computation/Charge Pump Input Energy Computation ==
  wEngine (rpm) : Inport
  tPump (N*m) : Inport  Port=2
  dispPump (cm^3/rev) : Inport  Port=3
  Abs : Abs  ZeroCross=off  SaturateOnIntegerOverflow=off
  Add : Sum
  Add1 : Sum
  Constant : Constant  Value=0
  Constant1 : Constant  Value=0
  Forward Gear : Switch  SaturateOnIntegerOverflow=off  InputSameDT=off
  Gain : Gain  Gain=2*pi/60
  Integrator : Integrator
  Integrator1 : Integrator
  Product : Product
  Reverse Gear : Switch  SaturateOnIntegerOverflow=off  InputSameDT=off
  convert to kW : Gain  Gain=1e-3
  Input Energy : Outport
  Input Power : Outport  Port=2
  wires:
  convert to kW/1 -> Reverse Gear/3, Forward Gear/1
  Abs/1 -> convert to kW/1
  Product/1 -> Abs/1
  Add/1 -> Input Energy/1  "Charge Pump Total Input Energy"
  Integrator/1 -> Add/2  "Pump Input Energy Forward Gear"
  Integrator1/1 -> Add/1  "Pump Input Energy Reverse Gear"
  Forward Gear/1 -> Add1/2, Integrator/1
  Reverse Gear/1 -> Add1/1, Integrator1/1
  Constant1/1 -> Forward Gear/3
  Constant/1 -> Reverse Gear/1
  dispPump (cm^3/rev)/1 -> Reverse Gear/2, Forward Gear/2
  wEngine (rpm)/1 -> Gain/1
  tPump (N*m)/1 -> Product/2
  Gain/1 -> Product/1
  Add1/1 -> Input Power/1  "Charge Pump Total Input Power"

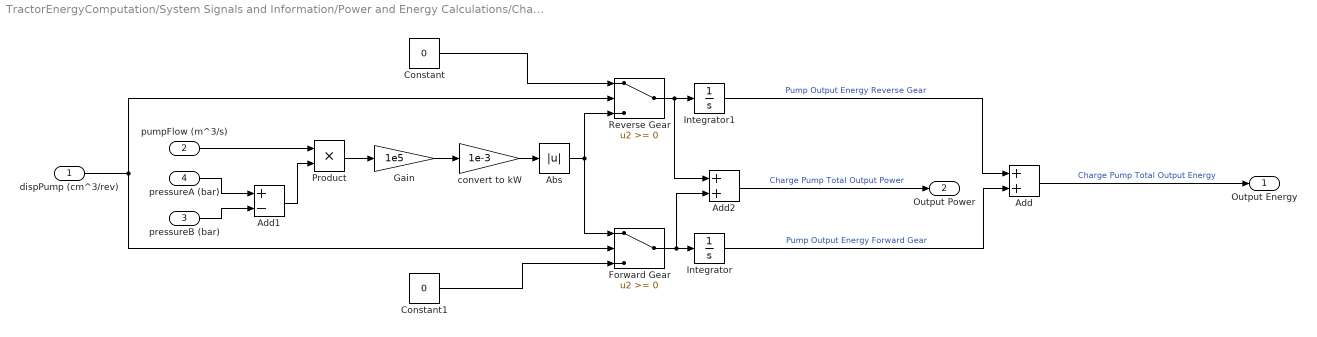
== system TractorEnergyComputation/System Signals and Information/Power and Energy Calculations/Charge Pump Computation/Charge Pump Output Energy Computation ==
  dispPump (cm^3/rev) : Inport
  pumpFlow (m^3/s) : Inport  Port=2
  pressureB (bar) : Inport  Port=3
  pressureA (bar) : Inport  Port=4
  Abs : Abs  ZeroCross=off  SaturateOnIntegerOverflow=off
  Add : Sum
  Add1 : Sum  Inputs=+-
  Add2 : Sum
  Constant : Constant  Value=0
  Constant1 : Constant  Value=0
  Forward Gear : Switch  SaturateOnIntegerOverflow=off  InputSameDT=off
  Gain : Gain  Gain=1e5
  Integrator : Integrator
  Integrator1 : Integrator
  Product : Product
  Reverse Gear : Switch  SaturateOnIntegerOverflow=off  InputSameDT=off
  convert to kW : Gain  Gain=1e-3
  Output Energy : Outport
  Output Power : Outport  Port=2
  wires:
  convert to kW/1 -> Abs/1
  Abs/1 -> Reverse Gear/3, Forward Gear/1
  Gain/1 -> convert to kW/1
  Add1/1 -> Product/2
  pressureB (bar)/1 -> Add1/2
  pressureA (bar)/1 -> Add1/1
  Add/1 -> Output Energy/1  "Charge Pump Total Output Energy"
  Integrator/1 -> Add/2  "Pump Output Energy Forward Gear"
  Integrator1/1 -> Add/1  "Pump Output Energy Reverse Gear"
  Forward Gear/1 -> Add2/2, Integrator/1
  Reverse Gear/1 -> Integrator1/1, Add2/1
  Constant1/1 -> Forward Gear/3
  Constant/1 -> Reverse Gear/1
  dispPump (cm^3/rev)/1 -> Forward Gear/2, Reverse Gear/2
  Product/1 -> Gain/1
  pumpFlow (m^3/s)/1 -> Product/1
  Add2/1 -> Output Power/1  "Charge Pump Total Output Power"

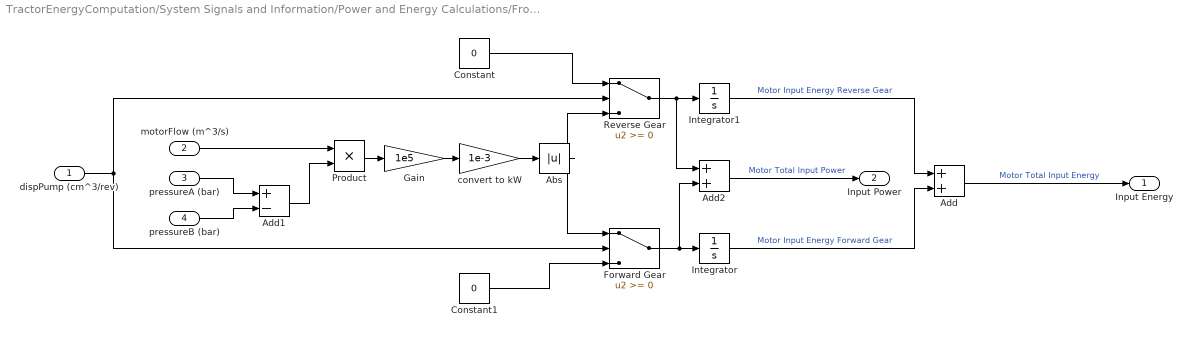
== system TractorEnergyComputation/System Signals and Information/Power and Energy Calculations/Front Motor Computation/Motor Input Energy Computation ==
  dispPump (cm^3/rev) : Inport
  motorFlow (m^3/s) : Inport  Port=2
  pressureA (bar) : Inport  Port=3
  pressureB (bar) : Inport  Port=4
  Abs : Abs  SaturateOnIntegerOverflow=off
  Add : Sum
  Add1 : Sum  Inputs=+-
  Add2 : Sum
  Constant : Constant  Value=0
  Constant1 : Constant  Value=0
  Forward Gear : Switch  SaturateOnIntegerOverflow=off  InputSameDT=off
  Gain : Gain  Gain=1e5
  Integrator : Integrator
  Integrator1 : Integrator
  Product : Product
  Reverse Gear : Switch  SaturateOnIntegerOverflow=off  InputSameDT=off
  convert to kW : Gain  Gain=1e-3
  "Input Energy " : Outport
  Input Power : Outport  Port=2
  wires:
  convert to kW/1 -> Abs/1
  Gain/1 -> convert to kW/1
  Abs/1 -> Reverse Gear/3, Forward Gear/1
  Add1/1 -> Product/2
  pressureB (bar)/1 -> Add1/2
  pressureA (bar)/1 -> Add1/1
  Add/1 -> "Input Energy "/1  "Motor Total Input Energy"
  Integrator/1 -> Add/2  "Motor Input Energy Forward Gear"
  Integrator1/1 -> Add/1  "Motor Input Energy Reverse Gear"
  Forward Gear/1 -> Add2/2, Integrator/1
  Constant1/1 -> Forward Gear/3
  Constant/1 -> Reverse Gear/1
  dispPump (cm^3/rev)/1 -> Reverse Gear/2, Forward Gear/2
  Product/1 -> Gain/1
  motorFlow (m^3/s)/1 -> Product/1
  Reverse Gear/1 -> Integrator1/1, Add2/1
  Add2/1 -> Input Power/1  "Motor Total Input Power"

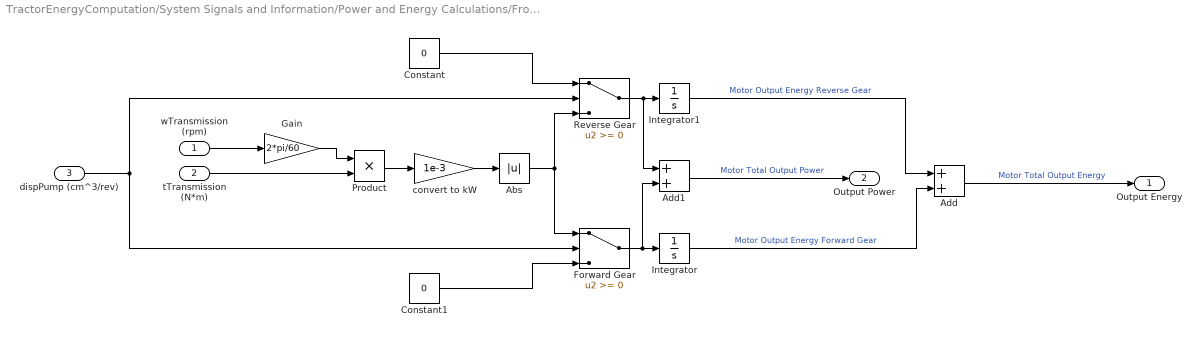
== system TractorEnergyComputation/System Signals and Information/Power and Energy Calculations/Front Motor Computation/Motor Output Energy Computation ==
  wTransmission (rpm) : Inport
  tTransmission (N*m) : Inport  Port=2
  dispPump (cm^3/rev) : Inport  Port=3
  Abs : Abs  ZeroCross=off  SaturateOnIntegerOverflow=off
  Add : Sum
  Add1 : Sum
  Constant : Constant  Value=0
  Constant1 : Constant  Value=0
  Forward Gear : Switch  SaturateOnIntegerOverflow=off  InputSameDT=off
  Gain : Gain  Gain=2*pi/60
  Integrator : Integrator
  Integrator1 : Integrator
  Product : Product
  Reverse Gear : Switch  SaturateOnIntegerOverflow=off  InputSameDT=off
  convert to kW : Gain  Gain=1e-3
  Output Energy : Outport
  Output Power : Outport  Port=2
  wires:
  convert to kW/1 -> Abs/1
  Abs/1 -> Reverse Gear/3, Forward Gear/1
  Product/1 -> convert to kW/1
  Add/1 -> Output Energy/1  "Motor Total Output Energy"
  Integrator/1 -> Add/2  "Motor Output Energy Forward Gear"
  Integrator1/1 -> Add/1  "Motor Output Energy Reverse Gear"
  Forward Gear/1 -> Add1/2, Integrator/1
  Reverse Gear/1 -> Integrator1/1, Add1/1
  Constant1/1 -> Forward Gear/3
  Constant/1 -> Reverse Gear/1
  dispPump (cm^3/rev)/1 -> Forward Gear/2, Reverse Gear/2
  wTransmission (rpm)/1 -> Gain/1
  tTransmission (N*m)/1 -> Product/2
  Gain/1 -> Product/1
  Add1/1 -> Output Power/1  "Motor Total Output Power"

== system TractorEnergyComputation/System Signals and Information/Power and Energy Calculations/Pump Computation/Pump Input Energy Computation ==
  wEngine (rpm) : Inport
  tPump (N*m) : Inport  Port=2
  dispPump (cm^3/rev) : Inport  Port=3
  Abs : Abs  ZeroCross=off  SaturateOnIntegerOverflow=off
  Add : Sum
  Add1 : Sum
  Constant : Constant  Value=0
  Constant1 : Constant  Value=0
  Forward Gear : Switch  SaturateOnIntegerOverflow=off  InputSameDT=off
  Gain : Gain  Gain=2*pi/60
  Integrator : Integrator
  Integrator1 : Integrator
  Product : Product
  Reverse Gear : Switch  SaturateOnIntegerOverflow=off  InputSameDT=off
  convert to kW : Gain  Gain=1e-3
  Input Energy : Outport
  Input Power : Outport  Port=2
  wires:
  Gain/1 -> Product/1
  tPump (N*m)/1 -> Product/2
  wEngine (rpm)/1 -> Gain/1
  dispPump (cm^3/rev)/1 -> Forward Gear/2, Reverse Gear/2
  Constant/1 -> Reverse Gear/1
  Constant1/1 -> Forward Gear/3
  Reverse Gear/1 -> Integrator1/1, Add1/1
  Forward Gear/1 -> Integrator/1, Add1/2
  Integrator1/1 -> Add/1  "Pump Input Energy Reverse Gear"
  Integrator/1 -> Add/2  "Pump Input Energy Forward Gear"
  Add/1 -> Input Energy/1  "Pump Total Input Energy"
  Product/1 -> Abs/1
  Abs/1 -> convert to kW/1
  convert to kW/1 -> Forward Gear/1, Reverse Gear/3
  Add1/1 -> Input Power/1  "Pump Total Input Power"

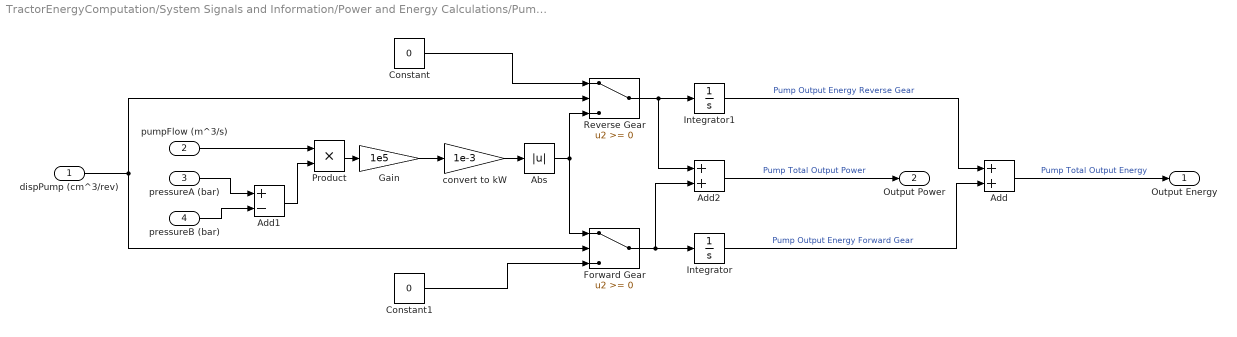
== system TractorEnergyComputation/System Signals and Information/Power and Energy Calculations/Pump Computation/Pump Output Energy Computation ==
  dispPump (cm^3/rev) : Inport
  pumpFlow (m^3/s) : Inport  Port=2
  pressureA (bar) : Inport  Port=3
  pressureB (bar) : Inport  Port=4
  Abs : Abs  ZeroCross=off  SaturateOnIntegerOverflow=off
  Add : Sum
  Add1 : Sum  Inputs=+-
  Add2 : Sum
  Constant : Constant  Value=0
  Constant1 : Constant  Value=0
  Forward Gear : Switch  SaturateOnIntegerOverflow=off  InputSameDT=off
  Gain : Gain  Gain=1e5
  Integrator : Integrator
  Integrator1 : Integrator
  Product : Product
  Reverse Gear : Switch  SaturateOnIntegerOverflow=off  InputSameDT=off
  convert to kW : Gain  Gain=1e-3
  Output Energy : Outport
  Output Power : Outport  Port=2
  wires:
  pumpFlow (m^3/s)/1 -> Product/1
  Product/1 -> Gain/1
  dispPump (cm^3/rev)/1 -> Reverse Gear/2, Forward Gear/2
  Constant/1 -> Reverse Gear/1
  Constant1/1 -> Forward Gear/3
  Reverse Gear/1 -> Integrator1/1, Add2/1
  Forward Gear/1 -> Integrator/1, Add2/2
  Integrator1/1 -> Add/1  "Pump Output Energy Reverse Gear"
  Integrator/1 -> Add/2  "Pump Output Energy Forward Gear"
  Add/1 -> Output Energy/1  "Pump Total Output Energy"
  pressureA (bar)/1 -> Add1/1
  pressureB (bar)/1 -> Add1/2
  Add1/1 -> Product/2
  Gain/1 -> convert to kW/1
  Abs/1 -> Forward Gear/1, Reverse Gear/3
  convert to kW/1 -> Abs/1
  Add2/1 -> Output Power/1  "Pump Total Output Power"

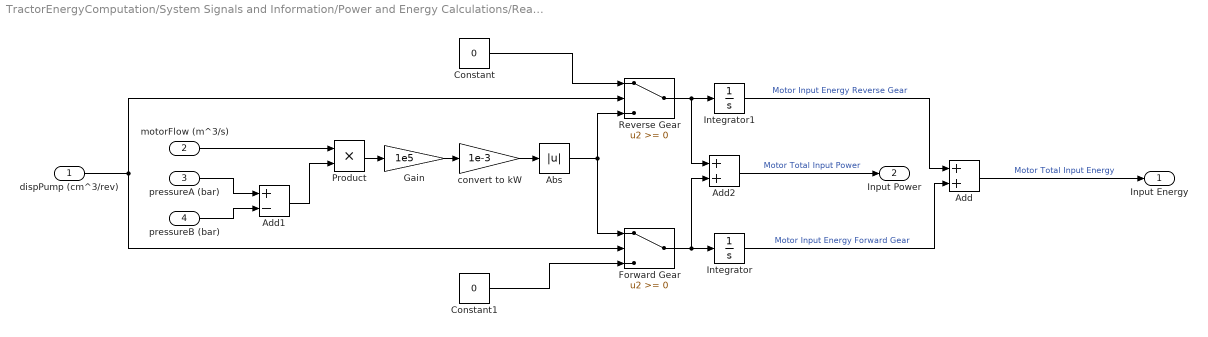
== system TractorEnergyComputation/System Signals and Information/Power and Energy Calculations/Rear Motor Computation/Motor Input Energy Computation ==
  dispPump (cm^3/rev) : Inport
  motorFlow (m^3/s) : Inport  Port=2
  pressureA (bar) : Inport  Port=3
  pressureB (bar) : Inport  Port=4
  Abs : Abs  SaturateOnIntegerOverflow=off
  Add : Sum
  Add1 : Sum  Inputs=+-
  Add2 : Sum
  Constant : Constant  Value=0
  Constant1 : Constant  Value=0
  Forward Gear : Switch  SaturateOnIntegerOverflow=off  InputSameDT=off
  Gain : Gain  Gain=1e5
  Integrator : Integrator
  Integrator1 : Integrator
  Product : Product
  Reverse Gear : Switch  SaturateOnIntegerOverflow=off  InputSameDT=off
  convert to kW : Gain  Gain=1e-3
  "Input Energy " : Outport
  Input Power : Outport  Port=2
  wires:
  motorFlow (m^3/s)/1 -> Product/1
  Product/1 -> Gain/1
  dispPump (cm^3/rev)/1 -> Forward Gear/2, Reverse Gear/2
  Constant/1 -> Reverse Gear/1
  Constant1/1 -> Forward Gear/3
  Reverse Gear/1 -> Add2/1, Integrator1/1
  Forward Gear/1 -> Add2/2, Integrator/1
  Integrator1/1 -> Add/1  "Motor Input Energy Reverse Gear"
  Integrator/1 -> Add/2  "Motor Input Energy Forward Gear"
  Add/1 -> "Input Energy "/1  "Motor Total Input Energy"
  pressureA (bar)/1 -> Add1/1
  pressureB (bar)/1 -> Add1/2
  Add1/1 -> Product/2
  Abs/1 -> Forward Gear/1, Reverse Gear/3
  Gain/1 -> convert to kW/1
  convert to kW/1 -> Abs/1
  Add2/1 -> Input Power/1  "Motor Total Input Power"

== system TractorEnergyComputation/System Signals and Information/Power and Energy Calculations/Rear Motor Computation/Motor Output Energy Computation ==
  wTransmission (rpm) : Inport
  tTransmission (N*m) : Inport  Port=2
  dispPump (cm^3/rev) : Inport  Port=3
  Abs : Abs  ZeroCross=off  SaturateOnIntegerOverflow=off
  Add : Sum
  Add1 : Sum
  Constant : Constant  Value=0
  Constant1 : Constant  Value=0
  Forward Gear : Switch  SaturateOnIntegerOverflow=off  InputSameDT=off
  Gain : Gain  Gain=2*pi/60
  Integrator : Integrator
  Integrator1 : Integrator
  Product : Product
  Reverse Gear : Switch  SaturateOnIntegerOverflow=off  InputSameDT=off
  convert to kW : Gain  Gain=1e-3
  Output Energy : Outport
  Output Power : Outport  Port=2
  wires:
  Gain/1 -> Product/1
  tTransmission (N*m)/1 -> Product/2
  wTransmission (rpm)/1 -> Gain/1
  dispPump (cm^3/rev)/1 -> Reverse Gear/2, Forward Gear/2
  Constant/1 -> Reverse Gear/1
  Constant1/1 -> Forward Gear/3
  Reverse Gear/1 -> Add1/1, Integrator1/1
  Forward Gear/1 -> Add1/2, Integrator/1
  Integrator1/1 -> Add/1  "Motor Output Energy Reverse Gear"
  Integrator/1 -> Add/2  "Motor Output Energy Forward Gear"
  Add/1 -> Output Energy/1  "Motor Total Output Energy"
  Product/1 -> convert to kW/1
  Abs/1 -> Forward Gear/1, Reverse Gear/3
  convert to kW/1 -> Abs/1
  Add1/1 -> Output Power/1  "Motor Total Output Power"

== system TractorEnergyComputation/Tractor/Tractor Body and Powertrain/Speed Source - Engine/Sensor Engine ==
  MRRef : fl_lib/Mechanical/Rotational Elements/Mechanical Rotational Reference
  Motion Sensor : fl_lib/Mechanical/Mechanical Sensors/Ideal Rotational Motion Sensor  reference=foundation.enum.MeasurementReference.difference  acceleration_port=false  velocity_port=true  position_port=true  wrap_angle=simscape.enum.onoff.off  offset=0 rad
  PS Terminator : fl_lib/Physical Signals/Sinks/PS Terminator
  PS-Simulink Converter : nesl_utility/PS-Simulink Converter  PhysicalDomain=network_engine_domain  SubClassName=ps_output  LeftPortType=input  RightPortType=output  PseudoPeriodic=off  Frequencies=[]  VectorFormat=1-D array  Unit=rpm  AffineConversion=off
  PS2S : nesl_utility/PS-Simulink Converter  PhysicalDomain=network_engine_domain  SubClassName=ps_output  LeftPortType=input  RightPortType=output  PseudoPeriodic=off  Frequencies=[]  VectorFormat=1-D array  Unit=N*m  AffineConversion=off
  Torque Sensor : fl_lib/Mechanical/Mechanical Sensors/Ideal Torque Sensor
  A : PMIOPort  Side=Left
  B : PMIOPort  Port=2  Side=Right
  Bus Element Out : Outport  PortName=engine  Element=engineSpeed
  Bus Element Out1 : Outport  PortName=engine  Element=engineTorque
  wires:
  PS2S/1 -> Bus Element Out1/1
  PS-Simulink Converter/1 -> Bus Element Out/1
  connections:
  Torque Sensor/LConn1 -- A/RConn1 -- Motion Sensor/LConn1
  Motion Sensor/RConn2 -- PS-Simulink Converter/LConn1
  MRRef/LConn1 -- Motion Sensor/RConn1
  Torque Sensor/RConn2 -- PS2S/LConn1
  B/RConn1 -- Torque Sensor/RConn1
  Motion Sensor/RConn3 -- PS Terminator/LConn1
